simulink model "tema"  (R2024b)
settings: Solver=VariableStepAuto  StartTime=0.0  StopTime=10.0  RelTol=1e-3
values from neighbouring files (symbols this model uses):
  C = 0.001    [script.m]
  L = 0.5    [script.m]
  R = 10    [script.m]
settings Model: Creator=alex_  LastModifiedBy=alex_

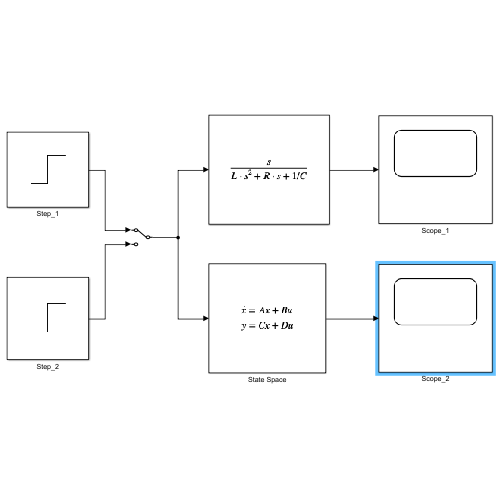
[thumbnail: Simulink's stored preview of the top-level diagram]
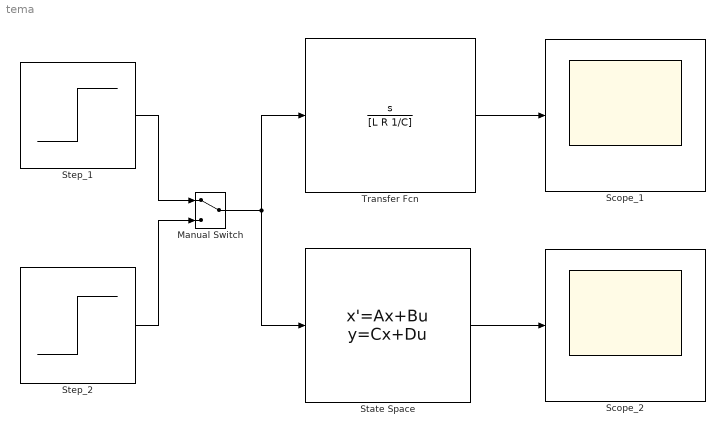
== system tema ==
  Manual Switch : ManualSwitch
  Scope_1 : Scope
  Scope_2 : Scope
  State Space : StateSpace  A=[0 1; -500 -5]  B=[0; 1]  C=[0 1]  D=0  InitialCondition=[0; 0]
  Step_1 : Step  Time=0  SampleTime=0
  Step_2 : Step  Time=0  After=2  SampleTime=0
  Transfer Fcn : TransferFcn  Numerator=[1 0]  Denominator=[L R 1/C]
  wires:
  Step_2/1 -> Manual Switch/2
  Step_1/1 -> Manual Switch/1
  Manual Switch/1 -> Transfer Fcn/1, State Space/1
  Transfer Fcn/1 -> Scope_1/1
  State Space/1 -> Scope_2/1
